simulink model "cable_driven_parallel_robot"  (R2023a)
settings: Solver=ode3  StartTime=0.0  StopTime=100  FixedStep=0.01  RelTol=1e-3
values from neighbouring files (symbols this model uses):
  cable_length = 1.2    [Model_Info.m]
  g = 9.81    [Model_Info.m]
  MP_H = 2    [Model_Info.m]
  MP_init_X = 0    [Model_Info.m]
  MP_init_Y = 0    [Model_Info.m]
  MP_init_Z = cable_length + (MP_H/2)    (= 2.2)    [Model_Info.m]
  MP_Ix = (MP_m/12)*(MP_W^2+MP_H^2)    (= 6.66666666667e-05)    [Model_Info.m]
  MP_Iy = (MP_m/12)*(MP_L^2+MP_H^2)    (= 6.66666666667e-05)    [Model_Info.m]
  MP_Iz = (MP_m/12)*(MP_L^2+MP_W^2)    (= 6.66666666667e-05)    [Model_Info.m]
  MP_L = 2    [Model_Info.m]
  MP_m = 0.0001    [Model_Info.m]
  MP_W = 2    [Model_Info.m]
  MR_init_X_L1 = -(MP_L/2)    (= -1)    [Model_Info.m]
  MR_init_X_L2 = (MP_L/2)    (= 1)    [Model_Info.m]
  MR_init_X_L3 = (MP_L/2)    (= 1)    [Model_Info.m]
  MR_init_X_L4 = -(MP_L/2)    (= -1)    [Model_Info.m]
  MR_init_Y_L1 = -(MP_W/2)    (= -1)    [Model_Info.m]
  MR_init_Y_L2 = -(MP_W/2)    (= -1)    [Model_Info.m]
  MR_init_Y_L3 = (MP_W/2)    (= 1)    [Model_Info.m]
  MR_init_Y_L4 = (MP_W/2)    (= 1)    [Model_Info.m]
  MR_init_Yaw_L1 = pi    (= 3.14159265359)    [Model_Info.m]
  MR_init_Yaw_L2 = 0    [Model_Info.m]
  MR_init_Yaw_L3 = 0    [Model_Info.m]
  MR_init_Yaw_L4 = pi    (= 3.14159265359)    [Model_Info.m]
  MR_Jr = (MR_m/12)*(MR_L^2+MR_W^2)    (= 0.333333333333)    [Model_Info.m]
  MR_m = 0.5    [Model_Info.m]
  MR_r = 2    [Model_Info.m]
  MR_WT = 2    [Model_Info.m]
  QR_Ax = 0.25*0    (= 0)    [Model_Info.m]
  QR_Ay = 0.25*0    (= 0)    [Model_Info.m]
  QR_Az = 0.25*0    (= 0)    [Model_Info.m]
  QR_b = 1.14*1e-7    (= 1.14e-07)    [Model_Info.m]
  QR_Ixx = 4.856*1e-3    (= 0.004856)    [Model_Info.m]
  QR_Iyy = 4.856*1e-3    (= 0.004856)    [Model_Info.m]
  QR_Izz = 8.801*1e-3    (= 0.008801)    [Model_Info.m]
  QR_K = 2.980*1e-6    (= 2.98e-06)    [Model_Info.m]
  QR_l = 0.225    [Model_Info.m]
  QR_m = 0.468    [Model_Info.m]
  QR_x0_U1 = -(MP_L/2)    (= -1)    [Model_Info.m]
  QR_x0_U2 = (MP_L/2)    (= 1)    [Model_Info.m]
  QR_x0_U3 = (MP_L/2)    (= 1)    [Model_Info.m]
  QR_x0_U4 = -(MP_L/2)    (= -1)    [Model_Info.m]
  QR_y0_U1 = -(MP_W/2)    (= -1)    [Model_Info.m]
  QR_y0_U2 = -(MP_W/2)    (= -1)    [Model_Info.m]
  QR_y0_U3 = (MP_W/2)    (= 1)    [Model_Info.m]
  QR_y0_U4 = (MP_W/2)    (= 1)    [Model_Info.m]
  QR_z0_U1 = 2*cable_length+(MP_H)    (= 4.4)    [Model_Info.m]
  QR_z0_U2 = 2*cable_length+(MP_H)    (= 4.4)    [Model_Info.m]
  QR_z0_U3 = 2*cable_length+(MP_H)    (= 4.4)    [Model_Info.m]
  QR_z0_U4 = 2*cable_length+(MP_H)    (= 4.4)    [Model_Info.m]
(part 2 of 12)

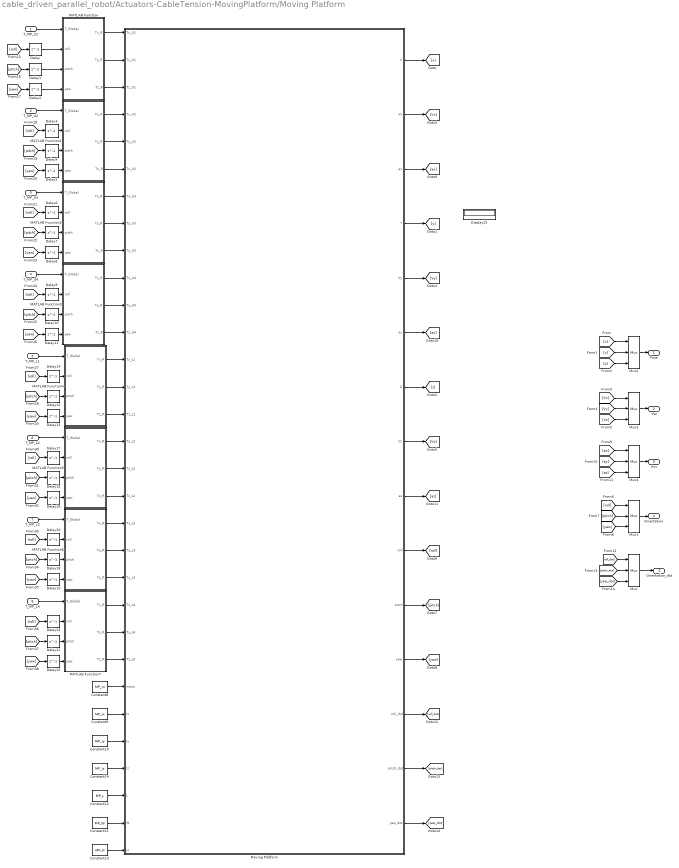
== system cable_driven_parallel_robot/Actuators-CableTension-MovingPlatform/Moving Platform ==
  T_MP_U1 : Inport
  "T_MP_U2 " : Inport  Port=2
  T_MP_U3 : Inport  Port=3
  T_MP_U4 : Inport  Port=4
  T_MP_L1 : Inport  Port=5
  T_MP_L2 : Inport  Port=6
  T_MP_L3 : Inport  Port=7
  T_MP_L4 : Inport  Port=8
  Constant10 : Constant  Value=MP_Iy
  Constant11 : Constant  Value=MP_W
  Constant12 : Constant  Value=MP_L
  Constant13 : Constant  Value=MP_H
  Constant14 : Constant  Value=MP_Iz
  Constant8 : Constant  Value=MP_m
  Constant9 : Constant  Value=MP_Ix
  Delay{,1..23} (24 alike) : Delay  DelayLength=1
  Display25 : Display
  MATLAB Function : MATLAB Function  TreatAsAtomicUnit=on
  MATLAB Function1 : MATLAB Function  TreatAsAtomicUnit=on
  MATLAB Function2 : MATLAB Function  TreatAsAtomicUnit=on
  MATLAB Function3 : MATLAB Function  TreatAsAtomicUnit=on
  MATLAB Function4 : MATLAB Function  TreatAsAtomicUnit=on
  MATLAB Function5 : MATLAB Function  TreatAsAtomicUnit=on
  MATLAB Function6 : MATLAB Function  TreatAsAtomicUnit=on
  MATLAB Function7 : MATLAB Function  TreatAsAtomicUnit=on
  Moving Platform : Subsystem
  Mux{,1..4} (5 alike) : Mux  Inputs=3
  Pose : Outport
  Vel : Outport  Port=2
  Acc : Outport  Port=3
  Orientation : Outport  Port=4
  Orientation_dot : Outport  Port=5
  wires:
  Constant14/1 -> Moving Platform/28(Iz)
  Constant10/1 -> Moving Platform/27(Iy)
  Constant11/1 -> Moving Platform/30(W)
  Constant9/1 -> Moving Platform/26(Ix)
  Constant13/1 -> Moving Platform/31(H)
  Constant12/1 -> Moving Platform/29(L)
  Constant8/1 -> Moving Platform/25(mass)
  [yaw] -> Mux1/3
  [roll] -> Mux1/1
  [pitch] -> Mux1/2
  [z] -> Mux2/3
  [Vx] -> Mux3/1
  [y] -> Mux2/2
  Mux/1 -> Orientation_dot/1
  [Vy] -> Mux3/2
  Mux1/1 -> Orientation/1
  [x] -> Mux2/1
  [roll_dot] -> Mux/1
  [ax] -> Mux4/1
  Mux4/1 -> Acc/1
  [az] -> Mux4/3
  [yaw_dot] -> Mux/3
  [Vz] -> Mux3/3
  [ay] -> Mux4/2
  Mux2/1 -> Pose/1
  Mux3/1 -> Vel/1
  [pitch_dot] -> Mux/2
  Moving Platform/7(Z) -> [z]
  Moving Platform/1(X) -> [x]
  Moving Platform/5(Vy) -> [Vy]
  Moving Platform/6(ay) -> [ay]
  Moving Platform/4(Y) -> [y]
  Moving Platform/2(Vx) -> [Vx]
  Moving Platform/3(ax) -> [ax]
  Moving Platform/9(az) -> [az]
  Moving Platform/8(Vz) -> [Vz]
  Moving Platform/12(yaw) -> [yaw]
  Moving Platform/11(pitch) -> [pitch]
  Moving Platform/15(yaw_dot) -> [yaw_dot]
  Moving Platform/14(pitch_dot) -> [pitch_dot]
  Moving Platform/10(roll) -> [roll]
  Moving Platform/13(roll_dot) -> [roll_dot]
  [roll] -> Delay/1
  Delay/1 -> MATLAB Function/2(roll)
  Delay1/1 -> MATLAB Function/3(pitch)
  [pitch] -> Delay1/1
  Delay2/1 -> MATLAB Function/4(yaw)
  [yaw] -> Delay2/1
  T_MP_U1/1 -> MATLAB Function/1(T_Global)
  MATLAB Function/2(Ty_R) -> Moving Platform/2(Ty_U1)
  MATLAB Function/3(Tz_R) -> Moving Platform/3(Tz_U1)
  Delay3/1 -> MATLAB Function1/2(roll)
  "T_MP_U2 "/1 -> MATLAB Function1/1(T_Global)
  Delay5/1 -> MATLAB Function1/4(yaw)
  [roll] -> Delay3/1
  [pitch] -> Delay4/1
  Delay4/1 -> MATLAB Function1/3(pitch)
  [yaw] -> Delay5/1
  MATLAB Function1/3(Tz_R) -> Moving Platform/6(Tz_U2)
  MATLAB Function1/2(Ty_R) -> Moving Platform/5(Ty_U2)
  MATLAB Function1/1(Tx_R) -> Moving Platform/4(Tx_U2)
  MATLAB Function2/1(Tx_R) -> Moving Platform/7(Tx_U3)
  MATLAB Function2/3(Tz_R) -> Moving Platform/9(Tz_U3)
  Delay7/1 -> MATLAB Function2/3(pitch)
  Delay6/1 -> MATLAB Function2/2(roll)
  [roll] -> Delay6/1
  Delay8/1 -> MATLAB Function2/4(yaw)
  [pitch] -> Delay7/1
  MATLAB Function2/2(Ty_R) -> Moving Platform/8(Ty_U3)
  T_MP_U3/1 -> MATLAB Function2/1(T_Global)
  [yaw] -> Delay8/1
  MATLAB Function3/1(Tx_R) -> Moving Platform/10(Tx_U4)
  MATLAB Function3/3(Tz_R) -> Moving Platform/12(Tz_U4)
  Delay10/1 -> MATLAB Function3/3(pitch)
  Delay9/1 -> MATLAB Function3/2(roll)
  [roll] -> Delay9/1
  Delay11/1 -> MATLAB Function3/4(yaw)
  [pitch] -> Delay10/1
  MATLAB Function3/2(Ty_R) -> Moving Platform/11(Ty_U4)
  T_MP_U4/1 -> MATLAB Function3/1(T_Global)
  [yaw] -> Delay11/1
  MATLAB Function4/1(Tx_R) -> Moving Platform/13(Tx_L1)
  MATLAB Function4/2(Ty_R) -> Moving Platform/14(Ty_L1)
  T_MP_L1/1 -> MATLAB Function4/1(T_Global)
  Delay13/1 -> MATLAB Function4/4(yaw)
  [roll] -> Delay14/1
  [yaw] -> Delay13/1
  Delay14/1 -> MATLAB Function4/2(roll)
  Delay12/1 -> MATLAB Function4/3(pitch)
  [pitch] -> Delay12/1
  MATLAB Function4/3(Tz_R) -> Moving Platform/15(Tz_L1)
  Delay15/1 -> MATLAB Function5/3(pitch)
  [roll] -> Delay17/1
  Delay16/1 -> MATLAB Function5/4(yaw)
  T_MP_L2/1 -> MATLAB Function5/1(T_Global)
  [yaw] -> Delay16/1
  [pitch] -> Delay15/1
  MATLAB Function5/2(Ty_R) -> Moving Platform/17(Ty_L2)
  MATLAB Function5/3(Tz_R) -> Moving Platform/18(Tz_L2)
  Delay17/1 -> MATLAB Function5/2(roll)
  MATLAB Function5/1(Tx_R) -> Moving Platform/16(Tx_L2)
  T_MP_L3/1 -> MATLAB Function6/1(T_Global)
  Delay19/1 -> MATLAB Function6/4(yaw)
  [roll] -> Delay20/1
  MATLAB Function6/1(Tx_R) -> Moving Platform/19(Tx_L3)
  Delay18/1 -> MATLAB Function6/3(pitch)
  MATLAB Function6/3(Tz_R) -> Moving Platform/21(Tz_L3)
  Delay20/1 -> MATLAB Function6/2(roll)
  MATLAB Function6/2(Ty_R) -> Moving Platform/20(Ty_L3)
  [pitch] -> Delay18/1
  [yaw] -> Delay19/1
  T_MP_L4/1 -> MATLAB Function7/1(T_Global)
  Delay22/1 -> MATLAB Function7/4(yaw)
  [roll] -> Delay23/1
  MATLAB Function7/1(Tx_R) -> Moving Platform/22(Tx_L4)
  Delay21/1 -> MATLAB Function7/3(pitch)
  MATLAB Function7/3(Tz_R) -> Moving Platform/24(Tz_L4)
  Delay23/1 -> MATLAB Function7/2(roll)
  MATLAB Function7/2(Ty_R) -> Moving Platform/23(Ty_L4)
  [pitch] -> Delay21/1
  [yaw] -> Delay22/1
  MATLAB Function/1(Tx_R) -> Moving Platform/1(Tx_U1)

== system cable_driven_parallel_robot/Actuators-CableTension-MovingPlatform/QuadRotor ==
  W1 : Inport
  W2 : Inport  Port=2
  W3 : Inport  Port=3
  W4 : Inport  Port=4
  T_U1_MP : Inport  Port=5
  Demux : Demux  Outputs=3
  Mux{,1..4} (5 alike) : Mux  Inputs=3
  QuadCopter Inputs : Subsystem
  Subsystem : Subsystem
  Pose : Outport
  Vel : Outport  Port=2
  Acc : Outport  Port=3
  Orientation : Outport  Port=4
  Orientation_dot : Outport  Port=5
  wires:
  QuadCopter Inputs/1(Integrated Inputs) -> Subsystem/1(Integrated Inputs)
  W3/1 -> QuadCopter Inputs/3(W3)
  W2/1 -> QuadCopter Inputs/2(W2)
  W1/1 -> QuadCopter Inputs/1(W1)
  W4/1 -> QuadCopter Inputs/4(W4)
  Subsystem/2(Vx) -> [Vx]
  Subsystem/5(Vy) -> [Vy]
  Subsystem/8(Vz) -> [Vz]
  Subsystem/10(Roll) -> [roll]
  Subsystem/11(Pitch) -> [pitch]
  Subsystem/12(Yaw) -> [yaw]
  Mux/1 -> Orientation_dot/1
  Mux1/1 -> Orientation/1
  Subsystem/4(Y) -> [y]
  Mux2/1 -> Pose/1
  Subsystem/7(Z) -> [z]
  Mux3/1 -> Vel/1
  Subsystem/1(X) -> [x]
  [x] -> Mux2/1
  [y] -> Mux2/2
  [z] -> Mux2/3
  [Vx] -> Mux3/1
  [Vy] -> Mux3/2
  [Vz] -> Mux3/3
  [roll] -> Mux1/1
  [pitch] -> Mux1/2
  [yaw] -> Mux1/3
  [ax] -> Mux4/1
  [az] -> Mux4/3
  Mux4/1 -> Acc/1
  [ay] -> Mux4/2
  [yaw_dot] -> Mux/3
  [roll_dot] -> Mux/1
  [pitch_dot] -> Mux/2
  Subsystem/3(ax) -> [ax]
  Subsystem/6(ay) -> [ay]
  Subsystem/9(az) -> [az]
  Subsystem/15(yaw_dot) -> [yaw_dot]
  Subsystem/14(pitch_dot) -> [pitch_dot]
  Subsystem/13(Roll_dot) -> [roll_dot]
  Demux/1 -> QuadCopter Inputs/5(Tx)
  Demux/2 -> QuadCopter Inputs/6(Ty)
  Demux/3 -> QuadCopter Inputs/7(Tz)
  T_U1_MP/1 -> Demux/1

== system cable_driven_parallel_robot/Actuators-CableTension-MovingPlatform/QuadRotor1 ==
  W1 : Inport
  W2 : Inport  Port=2
  W3 : Inport  Port=3
  W4 : Inport  Port=4
  T_U2_MP : Inport  Port=5
  Demux : Demux  Outputs=3
  Mux{,1..4} (5 alike) : Mux  Inputs=3
  QuadCopter Inputs : Subsystem
  Subsystem : Subsystem
  Pose : Outport
  Vel : Outport  Port=2
  Acc : Outport  Port=3
  Orientation : Outport  Port=4
  Orientation_dot : Outport  Port=5
  wires:
  T_U2_MP/1 -> Demux/1
  Demux/3 -> QuadCopter Inputs/7(Tz)
  Demux/2 -> QuadCopter Inputs/6(Ty)
  Demux/1 -> QuadCopter Inputs/5(Tx)
  Subsystem/13(Roll_dot) -> [roll_dot]
  Subsystem/14(pitch_dot) -> [pitch_dot]
  Subsystem/15(yaw_dot) -> [yaw_dot]
  Subsystem/9(az) -> [az]
  Subsystem/6(ay) -> [ay]
  Subsystem/3(ax) -> [ax]
  [pitch_dot] -> Mux/2
  [roll_dot] -> Mux/1
  [yaw_dot] -> Mux/3
  [ay] -> Mux4/2
  Mux4/1 -> Acc/1
  [az] -> Mux4/3
  [ax] -> Mux4/1
  [yaw] -> Mux1/3
  [pitch] -> Mux1/2
  [roll] -> Mux1/1
  [Vz] -> Mux3/3
  [Vy] -> Mux3/2
  [Vx] -> Mux3/1
  [z] -> Mux2/3
  [y] -> Mux2/2
  [x] -> Mux2/1
  Subsystem/1(X) -> [x]
  Mux3/1 -> Vel/1
  Subsystem/7(Z) -> [z]
  Mux2/1 -> Pose/1
  Subsystem/4(Y) -> [y]
  Mux1/1 -> Orientation/1
  Mux/1 -> Orientation_dot/1
  Subsystem/12(Yaw) -> [yaw]
  Subsystem/11(Pitch) -> [pitch]
  Subsystem/10(Roll) -> [roll]
  Subsystem/8(Vz) -> [Vz]
  Subsystem/5(Vy) -> [Vy]
  Subsystem/2(Vx) -> [Vx]
  W4/1 -> QuadCopter Inputs/4(W4)
  W1/1 -> QuadCopter Inputs/1(W1)
  W2/1 -> QuadCopter Inputs/2(W2)
  W3/1 -> QuadCopter Inputs/3(W3)
  QuadCopter Inputs/1(Integrated Inputs) -> Subsystem/1(Integrated Inputs)

== system cable_driven_parallel_robot/Actuators-CableTension-MovingPlatform/QuadRotor2 ==
  W1 : Inport
  W2 : Inport  Port=2
  W3 : Inport  Port=3
  W4 : Inport  Port=4
  T_U3_MP : Inport  Port=5
  Demux : Demux  Outputs=3
  Mux{,1..4} (5 alike) : Mux  Inputs=3
  QuadCopter Inputs : Subsystem
  Subsystem : Subsystem
  Pose : Outport
  Vel : Outport  Port=2
  Acc : Outport  Port=3
  Orientation : Outport  Port=4
  Orientation_dot : Outport  Port=5
  wires:
  QuadCopter Inputs/1(Integrated Inputs) -> Subsystem/1(Integrated Inputs)
  W3/1 -> QuadCopter Inputs/3(W3)
  W2/1 -> QuadCopter Inputs/2(W2)
  W1/1 -> QuadCopter Inputs/1(W1)
  W4/1 -> QuadCopter Inputs/4(W4)
  Subsystem/2(Vx) -> [Vx]
  Subsystem/5(Vy) -> [Vy]
  Subsystem/8(Vz) -> [Vz]
  Subsystem/10(Roll) -> [roll]
  Subsystem/11(Pitch) -> [pitch]
  Subsystem/12(Yaw) -> [yaw]
  Mux/1 -> Orientation_dot/1
  Mux1/1 -> Orientation/1
  Subsystem/4(Y) -> [y]
  Mux2/1 -> Pose/1
  Subsystem/7(Z) -> [z]
  Mux3/1 -> Vel/1
  Subsystem/1(X) -> [x]
  [x] -> Mux2/1
  [y] -> Mux2/2
  [z] -> Mux2/3
  [Vx] -> Mux3/1
  [Vy] -> Mux3/2
  [Vz] -> Mux3/3
  [roll] -> Mux1/1
  [pitch] -> Mux1/2
  [yaw] -> Mux1/3
  [ax] -> Mux4/1
  [az] -> Mux4/3
  Mux4/1 -> Acc/1
  [ay] -> Mux4/2
  [yaw_dot] -> Mux/3
  [roll_dot] -> Mux/1
  [pitch_dot] -> Mux/2
  Subsystem/3(ax) -> [ax]
  Subsystem/6(ay) -> [ay]
  Subsystem/9(az) -> [az]
  Subsystem/15(yaw_dot) -> [yaw_dot]
  Subsystem/14(pitch_dot) -> [pitch_dot]
  Subsystem/13(Roll_dot) -> [roll_dot]
  Demux/1 -> QuadCopter Inputs/5(Tx)
  Demux/2 -> QuadCopter Inputs/6(Ty)
  Demux/3 -> QuadCopter Inputs/7(Tz)
  T_U3_MP/1 -> Demux/1

== system cable_driven_parallel_robot/Actuators-CableTension-MovingPlatform/QuadRotor3 ==
  W1 : Inport
  W2 : Inport  Port=2
  W3 : Inport  Port=3
  W4 : Inport  Port=4
  T_U4_MP : Inport  Port=5
  Demux : Demux  Outputs=3
  Mux{,1..4} (5 alike) : Mux  Inputs=3
  QuadCopter Inputs : Subsystem
  Subsystem : Subsystem
  Pose : Outport
  Vel : Outport  Port=2
  Acc : Outport  Port=3
  Orientation : Outport  Port=4
  Orientation_dot : Outport  Port=5
  wires:
  T_U4_MP/1 -> Demux/1
  Demux/3 -> QuadCopter Inputs/7(Tz)
  Demux/2 -> QuadCopter Inputs/6(Ty)
  Demux/1 -> QuadCopter Inputs/5(Tx)
  Subsystem/13(Roll_dot) -> [roll_dot]
  Subsystem/14(pitch_dot) -> [pitch_dot]
  Subsystem/15(yaw_dot) -> [yaw_dot]
  Subsystem/9(az) -> [az]
  Subsystem/6(ay) -> [ay]
  Subsystem/3(ax) -> [ax]
  [pitch_dot] -> Mux/2
  [roll_dot] -> Mux/1
  [yaw_dot] -> Mux/3
  [ay] -> Mux4/2
  Mux4/1 -> Acc/1
  [az] -> Mux4/3
  [ax] -> Mux4/1
  [yaw] -> Mux1/3
  [pitch] -> Mux1/2
  [roll] -> Mux1/1
  [Vz] -> Mux3/3
  [Vy] -> Mux3/2
  [Vx] -> Mux3/1
  [z] -> Mux2/3
  [y] -> Mux2/2
  [x] -> Mux2/1
  Subsystem/1(X) -> [x]
  Mux3/1 -> Vel/1
  Subsystem/7(Z) -> [z]
  Mux2/1 -> Pose/1
  Subsystem/4(Y) -> [y]
  Mux1/1 -> Orientation/1
  Mux/1 -> Orientation_dot/1
  Subsystem/12(Yaw) -> [yaw]
  Subsystem/11(Pitch) -> [pitch]
  Subsystem/10(Roll) -> [roll]
  Subsystem/8(Vz) -> [Vz]
  Subsystem/5(Vy) -> [Vy]
  Subsystem/2(Vx) -> [Vx]
  W4/1 -> QuadCopter Inputs/4(W4)
  W1/1 -> QuadCopter Inputs/1(W1)
  W2/1 -> QuadCopter Inputs/2(W2)
  W3/1 -> QuadCopter Inputs/3(W3)
  QuadCopter Inputs/1(Integrated Inputs) -> Subsystem/1(Integrated Inputs)

== system cable_driven_parallel_robot/Input Managment/MR_Input_L1 ==
  1 : Constant  Value=0.1
  2 : Constant  Value=0.1
  TR_L1 : Outport
  TL_L1 : Outport  Port=2
  wires:
  2/1 -> TL_L1/1
  1/1 -> TR_L1/1

== system cable_driven_parallel_robot/Input Managment/MR_Input_L2 ==
  1 : Constant  Value=0.1
  2 : Constant  Value=0.1  VectorParams1D=off
  TR_L2 : Outport
  TL_L2 : Outport  Port=2
  wires:
  2/1 -> TL_L2/1
  1/1 -> TR_L2/1

== system cable_driven_parallel_robot/Input Managment/MR_Input_L3 ==
  1 : Constant  Value=0.1
  2 : Constant  Value=0.1
  TR_L3 : Outport
  TL_L3 : Outport  Port=2
  wires:
  2/1 -> TL_L3/1
  1/1 -> TR_L3/1

== system cable_driven_parallel_robot/Input Managment/MR_Input_L4 ==
  1 : Constant  Value=100
  2 : Constant  Value=100
  TR_L4 : Outport
  TL_L4 : Outport  Port=2
  wires:
  2/1 -> TL_L4/1
  1/1 -> TR_L4/1

== system cable_driven_parallel_robot/Input Managment/QR_Input_U1 ==
  1 : Constant  Value=607.1625
  2 : Constant  Value=638.2990
  3 : Constant  Value=607.1625
  4 : Constant  Value=638.2990
  W1_U1 : Outport
  W2_U1 : Outport  Port=2
  W3_U1 : Outport  Port=3
  W4_U1 : Outport  Port=4
  wires:
  2/1 -> W2_U1/1
  4/1 -> W4_U1/1
  1/1 -> W1_U1/1
  3/1 -> W3_U1/1

== system cable_driven_parallel_robot/Input Managment/QR_Input_U2 ==
  1 : Constant  Value=607.1625
  2 : Constant  Value=638.2990
  3 : Constant  Value=607.1625
  4 : Constant  Value=638.2990
  W1_U2 : Outport
  W2_U2 : Outport  Port=2
  W3_U2 : Outport  Port=3
  W4_U2 : Outport  Port=4
  wires:
  2/1 -> W2_U2/1
  4/1 -> W4_U2/1
  1/1 -> W1_U2/1
  3/1 -> W3_U2/1

== system cable_driven_parallel_robot/Input Managment/QR_Input_U3 ==
  1 : Constant  Value=607.1625
  2 : Constant  Value=638.2990
  3 : Constant  Value=607.1625
  4 : Constant  Value=638.2990
  W1_U3 : Outport
  W2_U3 : Outport  Port=2
  W3_U3 : Outport  Port=3
  W4_U3 : Outport  Port=4
  wires:
  2/1 -> W2_U3/1
  4/1 -> W4_U3/1
  1/1 -> W1_U3/1
  3/1 -> W3_U3/1

== system cable_driven_parallel_robot/Input Managment/QR_Input_U4 ==
  1 : Constant  Value=607.1625
  2 : Constant  Value=638.2990
  3 : Constant  Value=607.1625
  4 : Constant  Value=638.2990
  W1_U4 : Outport
  W2_U4 : Outport  Port=2
  W3_U4 : Outport  Port=3
  W4_U4 : Outport  Port=4
  wires:
  2/1 -> W2_U4/1
  4/1 -> W4_U4/1
  1/1 -> W1_U4/1
  3/1 -> W3_U4/1

== system cable_driven_parallel_robot/Target Wrench-Jacobian matrix/2 Wheels Diffrential Mobile Robot L1 ==
  TR_L1 : Inport
  TL_L1 : Inport  Port=2
  MP_Pose : Inport  Port=3
  MP_Orientation : Inport  Port=4
  "MR_Pose_L1 " : Inport  Port=5
  MR_Orientation_L1 : Inport  Port=6
  2 Wheels Diffrential Mobile Robot : Subsystem
  Constant : Constant  Value=MP_L
  Constant1 : Constant  Value=MP_W
  Constant18 : Constant  Value=MR_m
  Constant19 : Constant  Value=MR_r
  Constant2 : Constant  Value=MP_H
  Delay{1..3,16..18} (6 alike) : Delay  DelayLength=1
  Demux{,1..4} (5 alike) : Demux  Outputs=3
  IC1 : InitialCondition  Value=MP_init_X
  IC16 : InitialCondition  Value=0
  IC17 : InitialCondition  Value=0
  IC18 : InitialCondition  Value=0
  IC2 : InitialCondition  Value=MP_init_Y
  IC3 : InitialCondition  Value=MP_init_Z
  Mux : Mux  Inputs=3
  Mux1 : Mux  Inputs=3
  Terminator : Terminator
  Terminator1 : Terminator
  Transform : MATLAB Function  TreatAsAtomicUnit=on
  MR_F_L1 : Outport
  "isTension_L1 " : Outport  Port=2
  wires:
  Constant19/1 -> 2 Wheels Diffrential Mobile Robot/4(r)
  Constant18/1 -> 2 Wheels Diffrential Mobile Robot/3(mass)
  TL_L1/1 -> 2 Wheels Diffrential Mobile Robot/2(TL)
  TR_L1/1 -> 2 Wheels Diffrential Mobile Robot/1(TR)
  Demux/3 -> 2 Wheels Diffrential Mobile Robot/5(yaw)
  "MR_Pose_L1 "/1 -> Demux1/1
  Demux1/1 -> 2 Wheels Diffrential Mobile Robot/6(x_diff)
  Demux1/2 -> 2 Wheels Diffrential Mobile Robot/7(y_diff)
  Demux1/3 -> 2 Wheels Diffrential Mobile Robot/8(z_diff)
  Demux2/3 -> 2 Wheels Diffrential Mobile Robot/11(z_point)
  Demux2/2 -> 2 Wheels Diffrential Mobile Robot/10(y_point)
  Demux2/1 -> 2 Wheels Diffrential Mobile Robot/9(x_point)
  Constant/1 -> Transform/7(L)
  Constant1/1 -> Transform/8(W)
  Constant2/1 -> Transform/9(H)
  MP_Orientation/1 -> Demux3/1
  MP_Pose/1 -> Demux4/1
  Transform/1(MP_L1_X) -> Mux/1
  Transform/2(MP_L1_Y) -> Mux/2
  Transform/3(MP_L1_Z) -> Mux/3
  Mux/1 -> [MP_Pose_L1]
  [MP_Pose_L1] -> Demux2/1
  MR_Orientation_L1/1 -> Demux/1
  2 Wheels Diffrential Mobile Robot/4(isTension) -> "isTension_L1 "/1
  2 Wheels Diffrential Mobile Robot/2(Fy) -> Mux1/2
  2 Wheels Diffrential Mobile Robot/3(Fz) -> Mux1/3
  2 Wheels Diffrential Mobile Robot/1(Fx) -> Mux1/1
  Mux1/1 -> MR_F_L1/1
  Demux3/3 -> Delay18/1
  Demux3/2 -> Delay17/1
  Demux3/1 -> Delay16/1
  Demux4/1 -> Delay1/1
  Demux4/2 -> Delay2/1
  Demux4/3 -> Delay3/1
  IC3/1 -> Transform/6(MP_Z)
  IC2/1 -> Transform/5(MP_Y)
  IC1/1 -> Transform/4(MP_X)
  Delay2/1 -> IC2/1
  IC16/1 -> Transform/1(roll)
  IC18/1 -> Transform/3(yaw)
  IC17/1 -> Transform/2(pitch)
  Delay18/1 -> IC18/1
  Delay17/1 -> IC17/1
  Delay3/1 -> IC3/1
  Delay1/1 -> IC1/1
  Delay16/1 -> IC16/1
  Demux/1 -> Terminator/1
  Demux/2 -> Terminator1/1

== system cable_driven_parallel_robot/Target Wrench-Jacobian matrix/2 Wheels Diffrential Mobile Robot L2 ==
  TR_L2 : Inport
  TL_L2 : Inport  Port=2
  MP_Pose : Inport  Port=3
  MP_Orientation : Inport  Port=4
  "MR_Pose_L2 " : Inport  Port=5
  MR_Orientation_L2 : Inport  Port=6
  2 Wheels Diffrential Mobile Robot : Subsystem
  Constant : Constant  Value=MP_L
  Constant1 : Constant  Value=MP_W
  Constant18 : Constant  Value=MR_m
  Constant19 : Constant  Value=MR_r
  Constant2 : Constant  Value=MP_H
  Delay{1..3,16..18} (6 alike) : Delay  DelayLength=1
  Demux{,1..4} (5 alike) : Demux  Outputs=3
  IC1 : InitialCondition  Value=MP_init_X
  IC16 : InitialCondition  Value=0
  IC17 : InitialCondition  Value=0
  IC18 : InitialCondition  Value=0
  IC2 : InitialCondition  Value=MP_init_Y
  IC3 : InitialCondition  Value=MP_init_Z
  Mux : Mux  Inputs=3
  Mux1 : Mux  Inputs=3
  Terminator : Terminator
  Terminator1 : Terminator
  Transform : MATLAB Function  TreatAsAtomicUnit=on
  MR_F_L2 : Outport
  "isTension_L2 " : Outport  Port=2
  wires:
  Demux2/1 -> 2 Wheels Diffrential Mobile Robot/9(x_point)
  Demux2/2 -> 2 Wheels Diffrential Mobile Robot/10(y_point)
  Demux2/3 -> 2 Wheels Diffrential Mobile Robot/11(z_point)
  Demux1/3 -> 2 Wheels Diffrential Mobile Robot/8(z_diff)
  Demux1/2 -> 2 Wheels Diffrential Mobile Robot/7(y_diff)
  Demux1/1 -> 2 Wheels Diffrential Mobile Robot/6(x_diff)
  "MR_Pose_L2 "/1 -> Demux1/1
  Demux/3 -> 2 Wheels Diffrential Mobile Robot/5(yaw)
  TR_L2/1 -> 2 Wheels Diffrential Mobile Robot/1(TR)
  TL_L2/1 -> 2 Wheels Diffrential Mobile Robot/2(TL)
  Constant18/1 -> 2 Wheels Diffrential Mobile Robot/3(mass)
  Constant19/1 -> 2 Wheels Diffrential Mobile Robot/4(r)
  Constant1/1 -> Transform/8(W)
  Transform/2(MP_L2_Y) -> Mux/2
  Transform/3(MP_L2_Z) -> Mux/3
  Transform/1(MP_L2_X) -> Mux/1
  MP_Pose/1 -> Demux4/1
  Constant2/1 -> Transform/9(H)
  MP_Orientation/1 -> Demux3/1
  Constant/1 -> Transform/7(L)
  Mux/1 -> [MP_Pose_L2]
  [MP_Pose_L2] -> Demux2/1
  MR_Orientation_L2/1 -> Demux/1
  2 Wheels Diffrential Mobile Robot/4(isTension) -> "isTension_L2 "/1
  Mux1/1 -> MR_F_L2/1
  2 Wheels Diffrential Mobile Robot/2(Fy) -> Mux1/2
  2 Wheels Diffrential Mobile Robot/1(Fx) -> Mux1/1
  2 Wheels Diffrential Mobile Robot/3(Fz) -> Mux1/3
  Demux3/3 -> Delay18/1
  Demux3/2 -> Delay17/1
  Demux3/1 -> Delay16/1
  Demux4/1 -> Delay1/1
  Demux4/2 -> Delay2/1
  Demux4/3 -> Delay3/1
  IC16/1 -> Transform/1(roll)
  IC18/1 -> Transform/3(yaw)
  IC17/1 -> Transform/2(pitch)
  Delay18/1 -> IC18/1
  Delay17/1 -> IC17/1
  Delay16/1 -> IC16/1
  Delay2/1 -> IC2/1
  IC2/1 -> Transform/5(MP_Y)
  Delay3/1 -> IC3/1
  IC3/1 -> Transform/6(MP_Z)
  IC1/1 -> Transform/4(MP_X)
  Delay1/1 -> IC1/1
  Demux/1 -> Terminator/1
  Demux/2 -> Terminator1/1

== system cable_driven_parallel_robot/Target Wrench-Jacobian matrix/2 Wheels Diffrential Mobile Robot L3 ==
  TR_L3 : Inport
  TL_L3 : Inport  Port=2
  MP_Pose : Inport  Port=3
  MP_Orientation : Inport  Port=4
  "MR_Pose_L3 " : Inport  Port=5
  MR_Orientation_L3 : Inport  Port=6
  2 Wheels Diffrential Mobile Robot : Subsystem
  Constant : Constant  Value=MP_L
  Constant1 : Constant  Value=MP_W
  Constant18 : Constant  Value=MR_m
  Constant19 : Constant  Value=MR_r
  Constant2 : Constant  Value=MP_H
  Delay{1..3,16..18} (6 alike) : Delay  DelayLength=1
  Demux{,1..4} (5 alike) : Demux  Outputs=3
  IC1 : InitialCondition  Value=MP_init_X
  IC16 : InitialCondition  Value=0
  IC17 : InitialCondition  Value=0
  IC18 : InitialCondition  Value=0
  IC2 : InitialCondition  Value=MP_init_Y
  IC3 : InitialCondition  Value=MP_init_Z
  Mux : Mux  Inputs=3
  Mux1 : Mux  Inputs=3
  Terminator1 : Terminator
  Terminator2 : Terminator
  Transform : MATLAB Function  TreatAsAtomicUnit=on
  MR_F_L3 : Outport
  "isTension_L3 " : Outport  Port=2
  wires:
  Constant19/1 -> 2 Wheels Diffrential Mobile Robot/4(r)
  Constant18/1 -> 2 Wheels Diffrential Mobile Robot/3(mass)
  TL_L3/1 -> 2 Wheels Diffrential Mobile Robot/2(TL)
  TR_L3/1 -> 2 Wheels Diffrential Mobile Robot/1(TR)
  Demux/3 -> 2 Wheels Diffrential Mobile Robot/5(yaw)
  "MR_Pose_L3 "/1 -> Demux1/1
  Demux1/1 -> 2 Wheels Diffrential Mobile Robot/6(x_diff)
  Demux1/2 -> 2 Wheels Diffrential Mobile Robot/7(y_diff)
  Demux1/3 -> 2 Wheels Diffrential Mobile Robot/8(z_diff)
  Demux2/3 -> 2 Wheels Diffrential Mobile Robot/11(z_point)
  Demux2/2 -> 2 Wheels Diffrential Mobile Robot/10(y_point)
  Demux2/1 -> 2 Wheels Diffrential Mobile Robot/9(x_point)
  Mux/1 -> [MP_Pose_L3]
  MP_Orientation/1 -> Demux3/1
  Constant/1 -> Transform/7(L)
  MP_Pose/1 -> Demux4/1
  Constant2/1 -> Transform/9(H)
  Transform/1(MP_L3_X) -> Mux/1
  Transform/2(MP_L3_Y) -> Mux/2
  Constant1/1 -> Transform/8(W)
  Transform/3(MP_L3_Z) -> Mux/3
  [MP_Pose_L3] -> Demux2/1
  MR_Orientation_L3/1 -> Demux/1
  2 Wheels Diffrential Mobile Robot/4(isTension) -> "isTension_L3 "/1
  Mux1/1 -> MR_F_L3/1
  2 Wheels Diffrential Mobile Robot/2(Fy) -> Mux1/2
  2 Wheels Diffrential Mobile Robot/1(Fx) -> Mux1/1
  2 Wheels Diffrential Mobile Robot/3(Fz) -> Mux1/3
  Demux3/3 -> Delay18/1
  Demux3/2 -> Delay17/1
  Demux3/1 -> Delay16/1
  Demux4/1 -> Delay1/1
  Demux4/2 -> Delay2/1
  Demux4/3 -> Delay3/1
  IC16/1 -> Transform/1(roll)
  IC18/1 -> Transform/3(yaw)
  IC17/1 -> Transform/2(pitch)
  Delay18/1 -> IC18/1
  Delay17/1 -> IC17/1
  Delay16/1 -> IC16/1
  Delay2/1 -> IC2/1
  IC2/1 -> Transform/5(MP_Y)
  Delay3/1 -> IC3/1
  IC3/1 -> Transform/6(MP_Z)
  IC1/1 -> Transform/4(MP_X)
  Delay1/1 -> IC1/1
  Demux/1 -> Terminator1/1
  Demux/2 -> Terminator2/1

== system cable_driven_parallel_robot/Target Wrench-Jacobian matrix/2 Wheels Diffrential Mobile Robot L4 ==
  TR_L4 : Inport
  TL_L4 : Inport  Port=2
  MP_Pose : Inport  Port=3
  MR_Orientation : Inport  Port=4
  "MR_Pose_L4 " : Inport  Port=5
  MR_Orientation_L4 : Inport  Port=6
  2 Wheels Diffrential Mobile Robot : Subsystem
  Constant : Constant  Value=MP_L
  Constant1 : Constant  Value=MP_W
  Constant18 : Constant  Value=MR_m
  Constant19 : Constant  Value=MR_r
  Constant2 : Constant  Value=MP_H
  Delay{1..3,16..18} (6 alike) : Delay  DelayLength=1
  Demux{,1..4} (5 alike) : Demux  Outputs=3
  IC1 : InitialCondition  Value=MP_init_X
  IC16 : InitialCondition  Value=0
  IC17 : InitialCondition  Value=0
  IC18 : InitialCondition  Value=0
  IC2 : InitialCondition  Value=MP_init_Y
  IC3 : InitialCondition  Value=MP_init_Z
  Mux : Mux  Inputs=3
  Mux1 : Mux  Inputs=3
  Terminator1 : Terminator
  Terminator2 : Terminator
  Transform : MATLAB Function  TreatAsAtomicUnit=on
  MR_F_L4 : Outport
  "isTension_L4 " : Outport  Port=2
  wires:
  Demux2/1 -> 2 Wheels Diffrential Mobile Robot/9(x_point)
  Demux2/2 -> 2 Wheels Diffrential Mobile Robot/10(y_point)
  Demux2/3 -> 2 Wheels Diffrential Mobile Robot/11(z_point)
  Demux1/3 -> 2 Wheels Diffrential Mobile Robot/8(z_diff)
  Demux1/2 -> 2 Wheels Diffrential Mobile Robot/7(y_diff)
  Demux1/1 -> 2 Wheels Diffrential Mobile Robot/6(x_diff)
  "MR_Pose_L4 "/1 -> Demux1/1
  Demux/3 -> 2 Wheels Diffrential Mobile Robot/5(yaw)
  TR_L4/1 -> 2 Wheels Diffrential Mobile Robot/1(TR)
  TL_L4/1 -> 2 Wheels Diffrential Mobile Robot/2(TL)
  Constant18/1 -> 2 Wheels Diffrential Mobile Robot/3(mass)
  Constant19/1 -> 2 Wheels Diffrential Mobile Robot/4(r)
  Constant1/1 -> Transform/8(W)
  Transform/2(MP_L4_Y) -> Mux/2
  Transform/1(MP_L4_X) -> Mux/1
  Transform/3(MP_L4_Z) -> Mux/3
  Constant/1 -> Transform/7(L)
  Constant2/1 -> Transform/9(H)
  MR_Orientation/1 -> Demux3/1
  Mux/1 -> [MP_Pose_L4]
  MP_Pose/1 -> Demux4/1
  [MP_Pose_L4] -> Demux2/1
  MR_Orientation_L4/1 -> Demux/1
  2 Wheels Diffrential Mobile Robot/4(isTension) -> "isTension_L4 "/1
  Mux1/1 -> MR_F_L4/1
  2 Wheels Diffrential Mobile Robot/2(Fy) -> Mux1/2
  2 Wheels Diffrential Mobile Robot/1(Fx) -> Mux1/1
  2 Wheels Diffrential Mobile Robot/3(Fz) -> Mux1/3
  Demux3/3 -> Delay18/1
  Demux3/2 -> Delay17/1
  Demux3/1 -> Delay16/1
  Demux4/1 -> Delay1/1
  Demux4/2 -> Delay2/1
  Demux4/3 -> Delay3/1
  IC16/1 -> Transform/1(roll)
  IC18/1 -> Transform/3(yaw)
  IC17/1 -> Transform/2(pitch)
  Delay18/1 -> IC18/1
  Delay17/1 -> IC17/1
  Delay16/1 -> IC16/1
  Delay2/1 -> IC2/1
  IC2/1 -> Transform/5(MP_Y)
  Delay3/1 -> IC3/1
  IC3/1 -> Transform/6(MP_Z)
  IC1/1 -> Transform/4(MP_X)
  Delay1/1 -> IC1/1
  Demux/1 -> Terminator1/1
  Demux/2 -> Terminator2/1

== system cable_driven_parallel_robot/Target Wrench-Jacobian matrix/Moving Platform ==
  Constant8 : Constant  Value=MP_m
  Moving Platform : Subsystem
  Mux1 : Mux  Inputs=3
  MP_F : Outport
  wires:
  Constant8/1 -> Moving Platform/1(mass)
  ? -> ?
  Mux1/1 -> MP_F/1
  Moving Platform/2(Fy) -> Mux1/2
  Moving Platform/1(Fx) -> Mux1/1
  Moving Platform/3(Fz) -> Mux1/3

== system cable_driven_parallel_robot/Target Wrench-Jacobian matrix/QuadRotor U1 ==
  W1 : Inport
  W2 : Inport  Port=2
  W3 : Inport  Port=3
  W4 : Inport  Port=4
  "QR_Vel_U1 " : Inport  Port=5
  "QR_Orientation_U1 " : Inport  Port=6
  "QR_Orientation_dot_U1 " : Inport  Port=7
  "QR_Pose_U1 " : Inport  Port=8
  MP_Pose : Inport  Port=9
  MP_Orientation : Inport  Port=10
  Constant : Constant  Value=0
  Constant1 : Constant  Value=0
  Constant2 : Constant  Value=MP_L
  Constant3 : Constant  Value=0
  Constant4 : Constant  Value=MP_W
  Constant5 : Constant  Value=MP_H
  Delay{1..3,16..18} (6 alike) : Delay  DelayLength=1
  Demux{1..7} (7 alike) : Demux  Outputs=3
  Force Generator : Subsystem
  IC1 : InitialCondition  Value=MP_init_X
  IC16 : InitialCondition  Value=0
  IC17 : InitialCondition  Value=0
  IC18 : InitialCondition  Value=0
  IC2 : InitialCondition  Value=MP_init_Y
  IC3 : InitialCondition  Value=MP_init_Z
  Mux : Mux  Inputs=3
  Mux1 : Mux  Inputs=3
  QuadCopter Inputs : Subsystem
  Transform : MATLAB Function  TreatAsAtomicUnit=on
  QR_F_U1 : Outport
  isTension_U1 : Outport  Port=2
  wires:
  QuadCopter Inputs/1(Integrated Inputs) -> Force Generator/16(Integrated Inputs)
  W3/1 -> QuadCopter Inputs/3(W3)
  W2/1 -> QuadCopter Inputs/2(W2)
  W1/1 -> QuadCopter Inputs/1(W1)
  W4/1 -> QuadCopter Inputs/4(W4)
  Constant3/1 -> QuadCopter Inputs/7(Tz)
  Constant1/1 -> QuadCopter Inputs/6(Ty)
  Constant/1 -> QuadCopter Inputs/5(Tx)
  Demux4/1 -> Force Generator/10(x_rotor)
  Demux4/3 -> Force Generator/12(z_rotor)
  Demux4/2 -> Force Generator/11(y_rotor)
  Demux5/1 -> Force Generator/13(x_point)
  Demux1/3 -> Force Generator/3(vz)
  "QR_Vel_U1 "/1 -> Demux1/1
  Demux1/2 -> Force Generator/2(vy)
  Demux1/1 -> Force Generator/1(vx)
  Demux2/2 -> Force Generator/8(pitch)
  Demux2/1 -> Force Generator/7(roll)
  "QR_Orientation_U1 "/1 -> Demux2/1
  Demux2/3 -> Force Generator/9(yaw)
  "QR_Orientation_dot_U1 "/1 -> Demux3/1
  Demux3/1 -> Force Generator/4(roll_dot)
  Demux3/2 -> Force Generator/5(pitch_dot)
  Demux3/3 -> Force Generator/6(yaw_dot)
  "QR_Pose_U1 "/1 -> Demux4/1
  Demux5/3 -> Force Generator/15(z_point)
  Demux5/2 -> Force Generator/14(y_point)
  Constant4/1 -> Transform/8(W)
  Transform/2(MP_U1_Y) -> Mux/2
  Transform/3(MP_U1_Z) -> Mux/3
  Transform/1(MP_U1_X) -> Mux/1
  MP_Pose/1 -> Demux7/1
  Constant5/1 -> Transform/9(H)
  MP_Orientation/1 -> Demux6/1
  Constant2/1 -> Transform/7(L)
  Mux/1 -> [MP_Pose_U1]
  [MP_Pose_U1] -> Demux5/1
  Force Generator/4(isTension) -> isTension_U1/1
  Force Generator/1(Fx) -> Mux1/1
  Force Generator/2(Fy) -> Mux1/2
  Force Generator/3(Fz) -> Mux1/3
  Mux1/1 -> QR_F_U1/1
  Demux6/3 -> Delay18/1
  Demux6/2 -> Delay17/1
  Demux6/1 -> Delay16/1
  Demux7/1 -> Delay1/1
  Demux7/2 -> Delay2/1
  Demux7/3 -> Delay3/1
  IC16/1 -> Transform/1(roll)
  IC18/1 -> Transform/3(yaw)
  IC17/1 -> Transform/2(pitch)
  Delay18/1 -> IC18/1
  Delay17/1 -> IC17/1
  Delay16/1 -> IC16/1
  Delay2/1 -> IC2/1
  IC2/1 -> Transform/5(MP_Y)
  Delay3/1 -> IC3/1
  IC3/1 -> Transform/6(MP_Z)
  IC1/1 -> Transform/4(MP_X)
  Delay1/1 -> IC1/1

== system cable_driven_parallel_robot/Target Wrench-Jacobian matrix/QuadRotor U2 ==
  W1 : Inport
  W2 : Inport  Port=2
  W3 : Inport  Port=3
  W4 : Inport  Port=4
  "QR_Vel_U2 " : Inport  Port=5
  "QR_Orientation_U2 " : Inport  Port=6
  "QR_Orientation_dot_U2 " : Inport  Port=7
  QR_Pose_U2 : Inport  Port=8
  MP_Pose : Inport  Port=9
  MP_Orientation : Inport  Port=10
  Constant : Constant  Value=0
  Constant1 : Constant  Value=0
  Constant2 : Constant  Value=MP_L
  Constant3 : Constant  Value=0
  Constant4 : Constant  Value=MP_W
  Constant5 : Constant  Value=MP_H
  Delay{1..3,16..18} (6 alike) : Delay  DelayLength=1
  Demux{1..7} (7 alike) : Demux  Outputs=3
  Force Generator : Subsystem
  IC1 : InitialCondition  Value=MP_init_X
  IC16 : InitialCondition  Value=0
  IC17 : InitialCondition  Value=0
  IC18 : InitialCondition  Value=0
  IC2 : InitialCondition  Value=MP_init_Y
  IC3 : InitialCondition  Value=MP_init_Z
  Mux : Mux  Inputs=3
  Mux1 : Mux  Inputs=3
  QuadCopter Inputs : Subsystem
  Transform : MATLAB Function  TreatAsAtomicUnit=on
  QR_F_U2 : Outport
  isTension_U2 : Outport  Port=2
  wires:
  QuadCopter Inputs/1(Integrated Inputs) -> Force Generator/16(Integrated Inputs)
  W3/1 -> QuadCopter Inputs/3(W3)
  W2/1 -> QuadCopter Inputs/2(W2)
  W1/1 -> QuadCopter Inputs/1(W1)
  W4/1 -> QuadCopter Inputs/4(W4)
  Constant3/1 -> QuadCopter Inputs/7(Tz)
  Constant1/1 -> QuadCopter Inputs/6(Ty)
  Constant/1 -> QuadCopter Inputs/5(Tx)
  Demux4/1 -> Force Generator/10(x_rotor)
  Demux4/3 -> Force Generator/12(z_rotor)
  Demux4/2 -> Force Generator/11(y_rotor)
  Demux5/1 -> Force Generator/13(x_point)
  Demux1/3 -> Force Generator/3(vz)
  "QR_Vel_U2 "/1 -> Demux1/1
  Demux1/2 -> Force Generator/2(vy)
  Demux1/1 -> Force Generator/1(vx)
  Demux2/2 -> Force Generator/8(pitch)
  Demux2/1 -> Force Generator/7(roll)
  "QR_Orientation_U2 "/1 -> Demux2/1
  Demux2/3 -> Force Generator/9(yaw)
  "QR_Orientation_dot_U2 "/1 -> Demux3/1
  Demux3/1 -> Force Generator/4(roll_dot)
  Demux3/2 -> Force Generator/5(pitch_dot)
  Demux3/3 -> Force Generator/6(yaw_dot)
  QR_Pose_U2/1 -> Demux4/1
  Demux5/3 -> Force Generator/15(z_point)
  Demux5/2 -> Force Generator/14(y_point)
  MP_Orientation/1 -> Demux6/1
  Constant2/1 -> Transform/7(L)
  Constant5/1 -> Transform/9(H)
  MP_Pose/1 -> Demux7/1
  Mux/1 -> [MP_Pose_U2]
  Transform/2(MP_U2_Y) -> Mux/2
  Constant4/1 -> Transform/8(W)
  Transform/3(MP_U2_Z) -> Mux/3
  Transform/1(MP_U2_X) -> Mux/1
  [MP_Pose_U2] -> Demux5/1
  Force Generator/4(isTension) -> isTension_U2/1
  Force Generator/2(Fy) -> Mux1/2
  Force Generator/3(Fz) -> Mux1/3
  Force Generator/1(Fx) -> Mux1/1
  Mux1/1 -> QR_F_U2/1
  Demux6/3 -> Delay18/1
  Demux6/2 -> Delay17/1
  Demux6/1 -> Delay16/1
  Demux7/1 -> Delay1/1
  Demux7/2 -> Delay2/1
  Demux7/3 -> Delay3/1
  IC16/1 -> Transform/1(roll)
  IC18/1 -> Transform/3(yaw)
  IC17/1 -> Transform/2(pitch)
  Delay18/1 -> IC18/1
  Delay17/1 -> IC17/1
  Delay16/1 -> IC16/1
  Delay2/1 -> IC2/1
  IC2/1 -> Transform/5(MP_Y)
  Delay3/1 -> IC3/1
  IC3/1 -> Transform/6(MP_Z)
  IC1/1 -> Transform/4(MP_X)
  Delay1/1 -> IC1/1

== system cable_driven_parallel_robot/Target Wrench-Jacobian matrix/QuadRotor U3 ==
  W1 : Inport
  W2 : Inport  Port=2
  W3 : Inport  Port=3
  W4 : Inport  Port=4
  "QR_Vel_U3 " : Inport  Port=5
  "QR_Orientation_U3 " : Inport  Port=6
  "QR_Orientation_dot_U3 " : Inport  Port=7
  "QR_Pose_U3 " : Inport  Port=8
  MP_Pose : Inport  Port=9
  MP_Orientation : Inport  Port=10
  Constant : Constant  Value=0
  Constant1 : Constant  Value=0
  Constant2 : Constant  Value=MP_L
  Constant3 : Constant  Value=0
  Constant4 : Constant  Value=MP_W
  Constant5 : Constant  Value=MP_H
  Delay{1..3,16..18} (6 alike) : Delay  DelayLength=1
  Demux{1..7} (7 alike) : Demux  Outputs=3
  Force Generator : Subsystem
  IC1 : InitialCondition  Value=MP_init_X
  IC16 : InitialCondition  Value=0
  IC17 : InitialCondition  Value=0
  IC18 : InitialCondition  Value=0
  IC2 : InitialCondition  Value=MP_init_Y
  IC3 : InitialCondition  Value=MP_init_Z
  Mux : Mux  Inputs=3
  Mux1 : Mux  Inputs=3
  QuadCopter Inputs : Subsystem
  Transform : MATLAB Function  TreatAsAtomicUnit=on
  QR_F_U3 : Outport
  isTension_U3 : Outport  Port=2
  wires:
  Demux5/2 -> Force Generator/14(y_point)
  Demux5/3 -> Force Generator/15(z_point)
  "QR_Pose_U3 "/1 -> Demux4/1
  Demux3/3 -> Force Generator/6(yaw_dot)
  Demux3/2 -> Force Generator/5(pitch_dot)
  Demux3/1 -> Force Generator/4(roll_dot)
  "QR_Orientation_dot_U3 "/1 -> Demux3/1
  Demux2/3 -> Force Generator/9(yaw)
  "QR_Orientation_U3 "/1 -> Demux2/1
  Demux2/1 -> Force Generator/7(roll)
  Demux2/2 -> Force Generator/8(pitch)
  Demux1/1 -> Force Generator/1(vx)
  Demux1/2 -> Force Generator/2(vy)
  "QR_Vel_U3 "/1 -> Demux1/1
  Demux1/3 -> Force Generator/3(vz)
  Demux5/1 -> Force Generator/13(x_point)
  Demux4/2 -> Force Generator/11(y_rotor)
  Demux4/3 -> Force Generator/12(z_rotor)
  Demux4/1 -> Force Generator/10(x_rotor)
  Constant/1 -> QuadCopter Inputs/5(Tx)
  Constant1/1 -> QuadCopter Inputs/6(Ty)
  Constant3/1 -> QuadCopter Inputs/7(Tz)
  W4/1 -> QuadCopter Inputs/4(W4)
  W1/1 -> QuadCopter Inputs/1(W1)
  W2/1 -> QuadCopter Inputs/2(W2)
  W3/1 -> QuadCopter Inputs/3(W3)
  QuadCopter Inputs/1(Integrated Inputs) -> Force Generator/16(Integrated Inputs)
  Mux/1 -> [MP_Pose_U3]
  Transform/2(MP_U3_Y) -> Mux/2
  Constant4/1 -> Transform/8(W)
  Transform/3(MP_U3_Z) -> Mux/3
  Constant5/1 -> Transform/9(H)
  Transform/1(MP_U3_X) -> Mux/1
  MP_Pose/1 -> Demux7/1
  MP_Orientation/1 -> Demux6/1
  Constant2/1 -> Transform/7(L)
  [MP_Pose_U3] -> Demux5/1
  Force Generator/4(isTension) -> isTension_U3/1
  Force Generator/2(Fy) -> Mux1/2
  Force Generator/3(Fz) -> Mux1/3
  Force Generator/1(Fx) -> Mux1/1
  Mux1/1 -> QR_F_U3/1
  Demux6/3 -> Delay18/1
  Demux6/2 -> Delay17/1
  Demux6/1 -> Delay16/1
  Demux7/1 -> Delay1/1
  Demux7/2 -> Delay2/1
  Demux7/3 -> Delay3/1
  IC16/1 -> Transform/1(roll)
  IC18/1 -> Transform/3(yaw)
  IC17/1 -> Transform/2(pitch)
  Delay18/1 -> IC18/1
  Delay17/1 -> IC17/1
  Delay16/1 -> IC16/1
  Delay2/1 -> IC2/1
  IC2/1 -> Transform/5(MP_Y)
  Delay3/1 -> IC3/1
  IC3/1 -> Transform/6(MP_Z)
  IC1/1 -> Transform/4(MP_X)
  Delay1/1 -> IC1/1

== system cable_driven_parallel_robot/Target Wrench-Jacobian matrix/QuadRotor U4 ==
  W1 : Inport
  W2 : Inport  Port=2
  W3 : Inport  Port=3
  W4 : Inport  Port=4
  "QR_Vel_U4 " : Inport  Port=5
  "QR_Orientation_U4 " : Inport  Port=6
  "QR_Orientation_dot_U4 " : Inport  Port=7
  "QR_Pose_U4 " : Inport  Port=8
  MP_Pose : Inport  Port=9
  MP_Orientation : Inport  Port=10
  Constant : Constant  Value=0
  Constant1 : Constant  Value=0
  Constant2 : Constant  Value=MP_L
  Constant3 : Constant  Value=0
  Constant4 : Constant  Value=MP_W
  Constant5 : Constant  Value=MP_H
  Delay{1..3,16..18} (6 alike) : Delay  DelayLength=1
  Demux{1..7} (7 alike) : Demux  Outputs=3
  Force Generator : Subsystem
  IC1 : InitialCondition  Value=MP_init_X
  IC16 : InitialCondition  Value=0
  IC17 : InitialCondition  Value=0
  IC18 : InitialCondition  Value=0
  IC2 : InitialCondition  Value=MP_init_Y
  IC3 : InitialCondition  Value=MP_init_Z
  Mux : Mux  Inputs=3
  Mux1 : Mux  Inputs=3
  QuadCopter Inputs : Subsystem
  Transform : MATLAB Function  TreatAsAtomicUnit=on
  QR_F_U4 : Outport
  isTension_U4 : Outport  Port=2
  wires:
  QuadCopter Inputs/1(Integrated Inputs) -> Force Generator/16(Integrated Inputs)
  W3/1 -> QuadCopter Inputs/3(W3)
  W2/1 -> QuadCopter Inputs/2(W2)
  W1/1 -> QuadCopter Inputs/1(W1)
  W4/1 -> QuadCopter Inputs/4(W4)
  Constant3/1 -> QuadCopter Inputs/7(Tz)
  Constant1/1 -> QuadCopter Inputs/6(Ty)
  Constant/1 -> QuadCopter Inputs/5(Tx)
  Demux4/1 -> Force Generator/10(x_rotor)
  Demux4/3 -> Force Generator/12(z_rotor)
  Demux4/2 -> Force Generator/11(y_rotor)
  Demux5/1 -> Force Generator/13(x_point)
  Demux1/3 -> Force Generator/3(vz)
  "QR_Vel_U4 "/1 -> Demux1/1
  Demux1/2 -> Force Generator/2(vy)
  Demux1/1 -> Force Generator/1(vx)
  Demux2/2 -> Force Generator/8(pitch)
  Demux2/1 -> Force Generator/7(roll)
  "QR_Orientation_U4 "/1 -> Demux2/1
  Demux2/3 -> Force Generator/9(yaw)
  "QR_Orientation_dot_U4 "/1 -> Demux3/1
  Demux3/1 -> Force Generator/4(roll_dot)
  Demux3/2 -> Force Generator/5(pitch_dot)
  Demux3/3 -> Force Generator/6(yaw_dot)
  "QR_Pose_U4 "/1 -> Demux4/1
  Demux5/3 -> Force Generator/15(z_point)
  Demux5/2 -> Force Generator/14(y_point)
  Constant2/1 -> Transform/7(L)
  MP_Orientation/1 -> Demux6/1
  Transform/1(MP_U4_X) -> Mux/1
  Constant5/1 -> Transform/9(H)
  MP_Pose/1 -> Demux7/1
  Transform/3(MP_U4_Z) -> Mux/3
  Constant4/1 -> Transform/8(W)
  Transform/2(MP_U4_Y) -> Mux/2
  Mux/1 -> [MP_Pose_U4]
  [MP_Pose_U4] -> Demux5/1
  Force Generator/4(isTension) -> isTension_U4/1
  Force Generator/2(Fy) -> Mux1/2
  Force Generator/3(Fz) -> Mux1/3
  Force Generator/1(Fx) -> Mux1/1
  Mux1/1 -> QR_F_U4/1
  Demux6/3 -> Delay18/1
  Demux6/2 -> Delay17/1
  Demux6/1 -> Delay16/1
  Demux7/1 -> Delay1/1
  Demux7/2 -> Delay2/1
  Demux7/3 -> Delay3/1
  IC16/1 -> Transform/1(roll)
  IC18/1 -> Transform/3(yaw)
  IC17/1 -> Transform/2(pitch)
  Delay18/1 -> IC18/1
  Delay17/1 -> IC17/1
  Delay16/1 -> IC16/1
  Delay2/1 -> IC2/1
  IC2/1 -> Transform/5(MP_Y)
  Delay3/1 -> IC3/1
  IC3/1 -> Transform/6(MP_Z)
  IC1/1 -> Transform/4(MP_X)
  Delay1/1 -> IC1/1
